simulink model "gnc_InputConditioning"  (R2026b)
settings: Solver=VariableStepAuto
values from neighbouring files (symbols this model uses):
  cmd = mcmd.cmd    [gnc_missionFSM.m]
  Ts = prm.Ts    [gnc_missionFSM.m]    (also in gnc_mpcPlantUpdate.m)
undefined symbols (not defined in the file or in its folder): cmd_seq, P
libraries: simulink x5
settings Model: Creator=aomar  LastModifiedBy=aomar

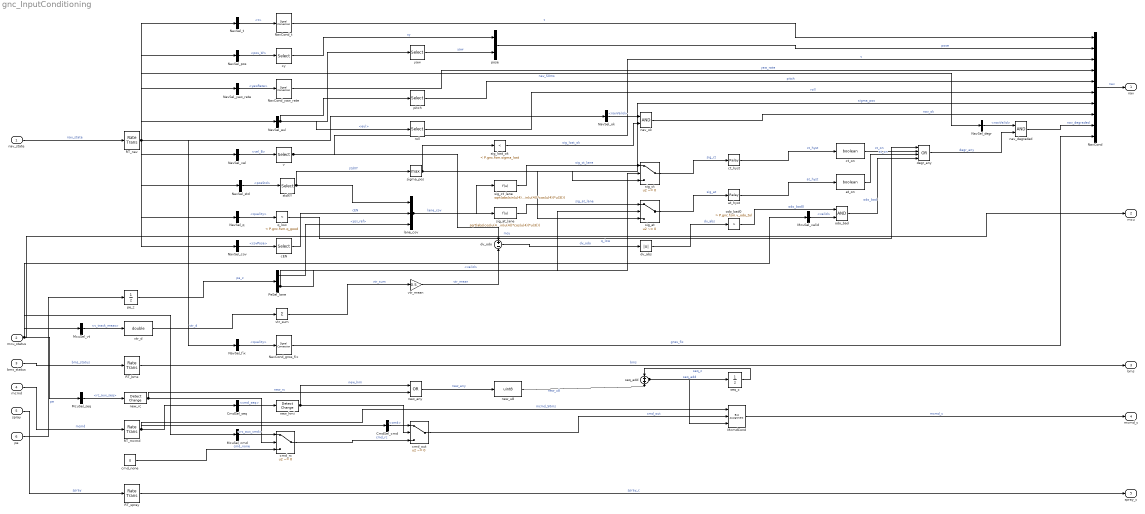
== system gnc_InputConditioning ==
  nav_state : Inport  OutDataTypeStr=Bus: Bus_NavState  SampleTime=Ts.nav
  mcu_status : Inport  Port=2  OutDataTypeStr=Bus: Bus_McuStatus  SampleTime=Ts.gnc
  bms_status : Inport  Port=3  OutDataTypeStr=Bus: Bus_BmsStatus  SampleTime=Ts.hk
  mcmd : Inport  Port=4  OutDataTypeStr=Bus: Bus_MissionCmd  SampleTime=Ts.mcmd
  spray : Inport  Port=5  OutDataTypeStr=Bus: Bus_SprayDemand  SampleTime=Ts.spray
  pe : Inport  Port=6  OutDataTypeStr=Bus: Bus_PathError  SampleTime=Ts.gnc
  CmdSel_cmd : BusSelector  OutputSignals=cmd
  CmdSel_seq : BusSelector  OutputSignals=cmd_seq
  McmdCond : BusAssignment  AssignedSignals=cmd,cmd_seq
  McuSel_cmd : BusSelector  OutputSignals=rc_aux_cmd
  McuSel_seq : BusSelector  OutputSignals=rc_aux_seq
  McuSel_valid : BusSelector  OutputSignals=valid
  McuSel_vt : BusSelector  OutputSignals=v_track_meas
  NavCond : BusCreator  Inputs=10  OutDataTypeStr=Bus: Bus_NavCond  NonVirtualBus=on
  NavCond_gnss_fix : SignalConversion  OverrideOpt=off
  NavCond_t : SignalConversion  OverrideOpt=off
  NavCond_yaw_rate : SignalConversion  OverrideOpt=off
  NavSel_cov : BusSelector  OutputSignals=covPose
  NavSel_degr : BusSelector  OutputSignals=navValid
  NavSel_eul : BusSelector  OutputSignals=eul
  NavSel_fix : BusSelector  OutputSignals=quality
  NavSel_ok : BusSelector  OutputSignals=navValid
  NavSel_pos : BusSelector  OutputSignals=pos_W
  NavSel_q : BusSelector  OutputSignals=quality
  NavSel_std : BusSelector  OutputSignals=posStd
  NavSel_t : BusSelector  OutputSignals=t
  NavSel_vel : BusSelector  OutputSignals=vel_B
  NavSel_yaw_rate : BusSelector  OutputSignals=yawRate
  PeSel_lane : BusSelector  OutputSignals=psi_ref,valid
  RT_bms : RateTransition  OutPortSampleTime=Ts.gnc
  RT_mcmd : RateTransition  OutPortSampleTime=Ts.gnc
  RT_nav : RateTransition  OutPortSampleTime=Ts.gnc
  RT_spray : RateTransition  OutPortSampleTime=Ts.gnc
  at_hyst : Relay  OnSwitchValue=P.gnc.fsm.sigma_along  OffSwitchValue=P.gnc.fsm.sigma_along_off  ZeroCross=off
  at_on : DataTypeConversion  OutDataTypeStr=boolean  RndMeth=Nearest
  cEN : Selector  NumberOfDimensions=2  InputPortWidth=3  IndexOptions=Index vector (dialog),Index vector (dialog)  Indices=1,2  OutputSizes=1
  cmd_none : Constant  Value=0  OutDataTypeStr=uint8  SampleTime=Ts.gnc
  cmd_out : Switch  Criteria=u2 ~= 0  SaturateOnIntegerOverflow=off  InputSameDT=off
  cmd_rc : Switch  Criteria=u2 ~= 0  SaturateOnIntegerOverflow=off  InputSameDT=off
  ct_hyst : Relay  OnSwitchValue=P.gnc.fsm.sigma_pause  OffSwitchValue=P.gnc.fsm.sigma_degr  ZeroCross=off
  ct_on : DataTypeConversion  OutDataTypeStr=boolean  RndMeth=Nearest
  degr_any : Logic  Operator=OR  Inputs=4  AllPortsSameDT=off  OutDataTypeStr=boolean
  dv_abs : Abs  SaturateOnIntegerOverflow=off
  dv_odo : Sum  Inputs=+-
  lane_cov : Mux  Inputs=3
  nav_degraded : Logic  AllPortsSameDT=off  OutDataTypeStr=boolean
  nav_ok : Logic  AllPortsSameDT=off  OutDataTypeStr=boolean
  new_any : Logic  Operator=OR  AllPortsSameDT=off  OutDataTypeStr=boolean
  new_hmi : simulink/Logic and Bit Operations/Detect Change  vinit=0  OutDataTypeStr=boolean
  new_rc : simulink/Logic and Bit Operations/Detect Change  vinit=0  OutDataTypeStr=boolean
  new_u8 : DataTypeConversion  OutDataTypeStr=uint8  RndMeth=Nearest
  odo_bad : Logic  AllPortsSameDT=off  OutDataTypeStr=boolean
  odo_bad0 : simulink/Logic and Bit Operations/Compare To Constant  relop=>  const=P.gnc.fsm.v_odo_tol  OutDataTypeStr=boolean
  pe_z : UnitDelay  InitialCondition=P.ic.Bus_PathError  SampleTime=-1
  pitch : Selector  IndexOptions=Index vector (dialog)  Indices=2  OutputSizes=1
  pose : Concatenate
  q_low : simulink/Logic and Bit Operations/Compare To Constant  relop=<  const=P.gnc.fsm.q_good  OutDataTypeStr=boolean
  roll : Selector  IndexOptions=Index vector (dialog)  Indices=3  OutputSizes=1
  seq_add : Sum  OutDataTypeStr=uint8
  seq_z : UnitDelay  InitialCondition=uint8(0)  SampleTime=-1
  sig_at : Switch  Criteria=u2 ~= 0  SaturateOnIntegerOverflow=off  InputSameDT=off
  sig_at_lane : Fcn  Expr=sqrt(abs(cos(u(4))^2*u(1)^2 + sin(u(4))^2*u(2)^2 + 2*sin(u(4))*cos(u(4))*u(3)))
  sig_ct : Switch  Criteria=u2 ~= 0  SaturateOnIntegerOverflow=off  InputSameDT=off
  sig_ct_lane : Fcn  Expr=sqrt(abs(sin(u(4))^2*u(1)^2 + cos(u(4))^2*u(2)^2 - 2*sin(u(4))*cos(u(4))*u(3)))
  sig_lost_ok : simulink/Logic and Bit Operations/Compare To Constant  relop=<  const=P.gnc.fsm.sigma_lost  OutDataTypeStr=boolean
  sigma_pos : MinMax  Function=max
  stdXY : Selector  IndexOptions=Index vector (dialog)  Indices=[1 2]  OutputSizes=1
  v : Selector  IndexOptions=Index vector (dialog)  Indices=1  OutputSizes=1
  vtr_d : DataTypeConversion  OutDataTypeStr=double  RndMeth=Nearest
  vtr_mean : Gain  Gain=0.5
  vtr_sum : Sum  Inputs=+
  xy : Selector  IndexOptions=Index vector (dialog)  Indices=[1 2]  OutputSizes=1
  yaw : Selector  IndexOptions=Index vector (dialog)  Indices=1  OutputSizes=1
  nav : Outport  OutDataTypeStr=Bus: Bus_NavCond
  mcu : Outport  Port=2  OutDataTypeStr=Bus: Bus_McuStatus
  bms : Outport  Port=3  OutDataTypeStr=Bus: Bus_BmsStatus
  mcmd_c : Outport  Port=4  OutDataTypeStr=Bus: Bus_MissionCmd
  spray_c : Outport  Port=5  OutDataTypeStr=Bus: Bus_SprayDemand
  wires:
  nav_state/1 -> RT_nav/1  "nav_state"
  mcu_status/1 -> mcu/1, McuSel_valid/1, McuSel_cmd/1, McuSel_seq/1, McuSel_vt/1  "mcu"
  bms_status/1 -> RT_bms/1  "bms_status"
  mcmd/1 -> RT_mcmd/1  "mcmd"
  spray/1 -> RT_spray/1  "spray"
  pe/1 -> pe_z/1  "pe"
  McuSel_vt/1 -> vtr_d/1  "<v_track_meas>"
  McuSel_seq/1 -> new_rc/1  "<rc_aux_seq>"
  cmd_none/1 -> cmd_rc/3  "cmd_none"
  pe_z/1 -> PeSel_lane/1  "pe_z"
  RT_nav/1 -> NavSel_fix/1, NavSel_t/1, NavSel_cov/1, NavSel_pos/1, NavSel_q/1, NavSel_yaw_rate/1, NavSel_std/1, NavSel_ok/1, NavSel_eul/1, NavSel_vel/1, NavSel_degr/1  "nav_50ms"
  RT_bms/1 -> bms/1  "bms"
  RT_mcmd/1 -> CmdSel_seq/1, McmdCond/1, CmdSel_cmd/1  "mcmd_50ms"
  RT_spray/1 -> spray_c/1  "spray_c"
  new_rc/1 -> cmd_rc/2, new_any/2  "new_rc"
  vtr_d/1 -> vtr_sum/1  "vtr_d"
  NavSel_t/1 -> NavCond_t/1  "<t>"
  NavSel_pos/1 -> xy/1  "<pos_W>"
  NavSel_yaw_rate/1 -> NavCond_yaw_rate/1  "<yawRate>"
  NavSel_vel/1 -> v/1  "<vel_B>"
  NavSel_q/1 -> q_low/1  "<quality>"
  NavSel_cov/1 -> cEN/1  "<covPose>"
  NavSel_fix/1 -> NavCond_gnss_fix/1  "<quality>"
  CmdSel_seq/1 -> new_hmi/1  "<cmd_seq>"
  McuSel_cmd/1 -> cmd_rc/1  "<rc_aux_cmd>"
  NavSel_std/1 -> stdXY/1  "<posStd>"
  NavSel_eul/1 -> yaw/1, pitch/1, roll/1  "<eul>"
  PeSel_lane/1 -> lane_cov/3  "<psi_ref>"
  PeSel_lane/2 -> sig_ct/2, sig_at/2  "<valid>"
  q_low/1 -> degr_any/1  "q_low"
  vtr_sum/1 -> vtr_mean/1  "vtr_sum"
  NavCond_t/1 -> NavCond/1  "t"
  xy/1 -> pose/1  "xy"
  NavCond_yaw_rate/1 -> NavCond/4  "yaw_rate"
  v/1 -> NavCond/3, dv_odo/1  "v"
  cEN/1 -> lane_cov/2  "cEN"
  NavCond_gnss_fix/1 -> NavCond/10  "gnss_fix"
  stdXY/1 -> lane_cov/1, sigma_pos/1  "stdXY"
  cmd_rc/1 -> cmd_out/3  "cmd_rc"
  new_hmi/1 -> cmd_out/2, new_any/1  "new_hmi"
  CmdSel_cmd/1 -> cmd_out/1  "<cmd>"
  lane_cov/1 -> sig_ct_lane/1, sig_at_lane/1  "lane_cov"
  sigma_pos/1 -> NavCond/7, sig_at/3, sig_lost_ok/1, sig_ct/3  "sigma_pos"
  vtr_mean/1 -> dv_odo/2  "vtr_mean"
  new_any/1 -> new_u8/1  "new_any"
  yaw/1 -> pose/2  "yaw"
  pitch/1 -> NavCond/5  "pitch"
  roll/1 -> NavCond/6  "roll"
  cmd_out/1 -> McmdCond/2  "cmd_out"
  pose/1 -> NavCond/2  "pose"
  dv_odo/1 -> dv_abs/1  "dv_odo"
  sig_lost_ok/1 -> nav_ok/2  "sig_lost_ok"
  sig_ct_lane/1 -> sig_ct/1  "sig_ct_lane"
  sig_at_lane/1 -> sig_at/1  "sig_at_lane"
  new_u8/1 -> seq_add/2  "new_u8"
  NavSel_ok/1 -> nav_ok/1  "<navValid>"
  seq_add/1 -> McmdCond/3, seq_z/1  "seq_add"
  nav_ok/1 -> NavCond/8  "nav_ok"
  dv_abs/1 -> odo_bad0/1  "dv_abs"
  sig_ct/1 -> ct_hyst/1  "sig_ct"
  sig_at/1 -> at_hyst/1  "sig_at"
  ct_hyst/1 -> ct_on/1  "ct_hyst"
  at_hyst/1 -> at_on/1  "at_hyst"
  odo_bad0/1 -> odo_bad/1  "odo_bad0"
  seq_z/1 -> seq_add/1  "seq_z"
  McmdCond/1 -> mcmd_c/1  "mcmd_c"
  McuSel_valid/1 -> odo_bad/2  "<valid>"
  odo_bad/1 -> degr_any/4  "odo_bad"
  ct_on/1 -> degr_any/2  "ct_on"
  at_on/1 -> degr_any/3  "at_on"
  degr_any/1 -> nav_degraded/2  "degr_any"
  NavSel_degr/1 -> nav_degraded/1  "<navValid>"
  nav_degraded/1 -> NavCond/9  "nav_degraded"
  NavCond/1 -> nav/1  "nav"
